simulink model "lab3Sim484"  (R2024a)
settings: Solver=VariableStepAuto  StartTime=0.0  StopTime=30.0  RelTol=1e-3
settings Model: Creator=pktubs  LastModifiedBy=pktubs

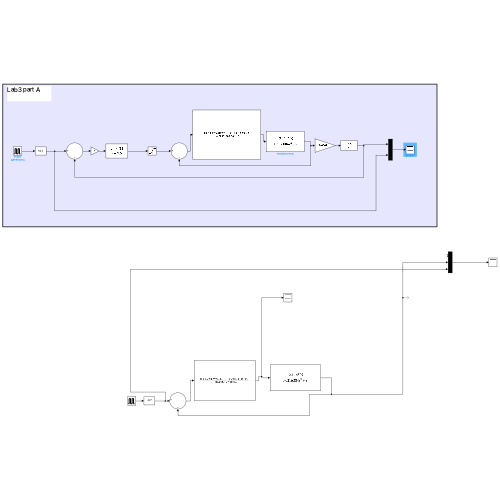
[thumbnail: Simulink's stored preview of the top-level diagram]
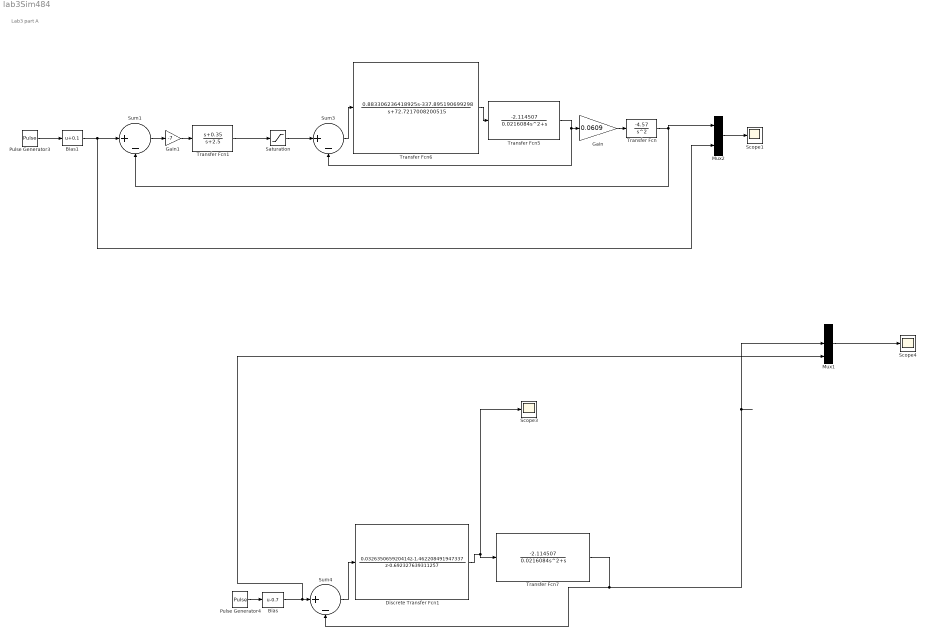
== system lab3Sim484 ==
  note: Lab3 part A
  Bias : Bias  Bias=-0.7  SaturateOnIntegerOverflow=off
  Bias1 : Bias  Bias=0.1  SaturateOnIntegerOverflow=off
  Discrete Transfer Fcn1 : DiscreteTransferFcn  Numerator=[0.032635065920414 -1.462208491947337]  Denominator=[1 -0.692327639311257]  SampleTime=0.005
  Gain : Gain  Gain=0.0609
  Gain1 : Gain  Gain=-7
  Mux1 : Mux  Inputs=3
  Mux2 : Mux  Inputs=2
  Pulse Generator3 : DiscretePulseGenerator  PulseType=Time based  Amplitude=0.15  Period=30  PulseWidth=50
  Pulse Generator4 : DiscretePulseGenerator  PulseType=Time based  Amplitude=1.4  PulseWidth=50
  Saturation : Saturate  UpperLimit=0.7  LowerLimit=-0.7
  Scope1 : Scope
  Scope3 : Scope
  Scope4 : Scope
  Sum1 : Sum  Inputs=|+-
  Sum3 : Sum  Inputs=|+-
  Sum4 : Sum  Inputs=|+-
  Transfer Fcn : TransferFcn  Numerator=[-4.57]  Denominator=[1 0 0]
  Transfer Fcn1 : TransferFcn  Numerator=[1 0.35]  Denominator=[1 2.5]
  Transfer Fcn5 : TransferFcn  Numerator=[-2.114507]  Denominator=[0.0216084 1 0]
  Transfer Fcn6 : TransferFcn  Numerator=[0.883306236418925 -337.895190699298]  Denominator=[1 72.7217008200515]
  Transfer Fcn7 : TransferFcn  Numerator=[-2.114507]  Denominator=[0.0216084 1 0]
  wires:
  Sum3/1 -> Transfer Fcn6/1
  Transfer Fcn6/1 -> Transfer Fcn5/1
  Transfer Fcn7/1 -> Sum4/2, Mux1/2
  Sum4/1 -> Discrete Transfer Fcn1/1
  Discrete Transfer Fcn1/1 -> Transfer Fcn7/1, Scope3/1
  Transfer Fcn5/1 -> Sum3/2, Gain/1
  Mux1/1 -> Scope4/1
  Pulse Generator4/1 -> Bias/1
  Bias/1 -> Mux1/3, Sum4/1
  Pulse Generator3/1 -> Bias1/1
  Gain/1 -> Transfer Fcn/1
  Transfer Fcn1/1 -> Saturation/1
  Gain1/1 -> Transfer Fcn1/1
  Bias1/1 -> Mux2/2, Sum1/1
  Sum1/1 -> Gain1/1
  Transfer Fcn/1 -> Sum1/2, Mux2/1
  Mux2/1 -> Scope1/1
  Saturation/1 -> Sum3/1
